simulink model "snap_adc5g_spec_rpi"  (R2019a)
settings: Solver=VariableStepDiscrete  StartTime=0.0  StopTime=10.0  RelTol=1e-3
undefined symbols (not defined in the file): pfb_coeff_gen_calc
libraries: xbsIndex_r4 x13965, casper_library_misc x80, casper_library_delays x43, xps_library x5, xbsReplacements_r4 x2, casper_library_communications x1
(part 36 of 152)

== system snap_adc5g_spec_rpi/fft_wideband_real/fft_direct/butterfly1_0/twiddle ==
  ai : Inport
  bi : Inport  Port=2
  sync_in : Inport  Port=3
  bus_convert : Subsystem  AncestorBlock=casper_library_bus/bus_convert  mask(bus_convert){n_bits_in=repmat(input_bit_width+coeff_bit_width+1, 1, n_inputs), bin_pt_in=(bin_pt_in+coeff_bit_width-1), cmplx=on, n_bits_out=input_bit_width+1, bin_pt_out=bin_pt_in, quantization=2, overflow=0, csp_latency=conv_latency, of=off, misc=on}
      mask prompts: n_bits_in "input bit widths"; bin_pt_in "input binary points"; cmplx "input complex"; n_bits_out "output bit widths"; bin_pt_out "output binary points"; quantization "quantization strategy (Truncate=0, Round  (unbiased: +/- Inf)=1, Round (unbiased: Even Values)=2)"; overflow "overflow strategy (Wrap=0, Saturate=1, Flag as error=2)"; csp_latency "latency"; of "overflow indication"; misc "misc support"
      mask help: Convert components of busses
      mask init: same as snap_adc5g_spec_rpi/fft_wideband_real/fft_direct/butterfly0_0/bus_convert
  bus_create : Subsystem  AncestorBlock=casper_library_flow_control/bus_create  mask(bus_create){inputNum=3}
      mask prompts: inputNum "Number of inputs:"
      mask init:
      | bus_create_init(gcb,...
      |     'inputNum', inputNum);
  bus_expand : Subsystem  AncestorBlock=casper_library_flow_control/bus_expand  mask(bus_expand){mode=divisions of arbitrary size, outputNum=1, outputWidth=[n_inputs*input_bit_width*2, 1+(n_inputs*input_bit_width*2)], outputBinaryPt=[0 0], outputArithmeticType=[0 0], show_format=off, outputToWorkspace=off, variablePrefix=out, outputToModelAsWell=on}
      mask prompts: outputNum "Number of outputs:"; outputWidth "Output width [msb ... lsb]:"; outputBinaryPt "Output binary point position [msb ... lsb]:"; outputArithmeticType "Output arithmetic type (ufix=0, fix=1, bool=2) [msb ... lsb]:"; show_format "Print format string?"; outputToWorkspace "Output to workspace?"; variablePrefix "Variable name prefix:"; outputToModelAsWell "Output to model as well?"
      mask help:
      | Expands a 'bus' made using a bus_create or Xilinx
      | concat block.
      | The input will be divided into the specified number
      | of outputs with the specified arithmetic types.
      | Divisions are made from most significant bit.
      mask init: same as snap_adc5g_spec_rpi/ss_adc/ctrl_split
      settings: AttributesFormatString=2 outputs
      mask TypeOptions mode: divisions of equal size | divisions of arbitrary size
      mask Callback mode: bus_expand_callback();
      mask Callback outputWidth: bus_expand_callback();
      mask Callback outputToWorkspace: bus_expand_callback();
  bus_expand1 : Subsystem  AncestorBlock=casper_library_flow_control/bus_expand  mask(bus_expand){mode=divisions of arbitrary size, outputNum=1, outputWidth=[1 72], outputBinaryPt=[0 0], outputArithmeticType=[2 0], show_format=off, outputToWorkspace=off, variablePrefix=out, outputToModelAsWell=on}
      mask prompts: outputNum "Number of outputs:"; outputWidth "Output width [msb ... lsb]:"; outputBinaryPt "Output binary point position [msb ... lsb]:"; outputArithmeticType "Output arithmetic type (ufix=0, fix=1, bool=2) [msb ... lsb]:"; show_format "Print format string?"; outputToWorkspace "Output to workspace?"; variablePrefix "Variable name prefix:"; outputToModelAsWell "Output to model as well?"
      mask help:
      | Expands a 'bus' made using a bus_create or Xilinx
      | concat block.
      | The input will be divided into the specified number
      | of outputs with the specified arithmetic types.
      | Divisions are made from most significant bit.
      mask init: same as snap_adc5g_spec_rpi/ss_adc/ctrl_split
      settings: AttributesFormatString=2 outputs
      mask TypeOptions mode: divisions of equal size | divisions of arbitrary size
      mask Callback mode: bus_expand_callback();
      mask Callback outputWidth: bus_expand_callback();
      mask Callback outputToWorkspace: bus_expand_callback();
  bus_mult : Subsystem  AncestorBlock=casper_library_bus/bus_mult  mask(bus_mult){n_bits_a=coeff_bit_width, bin_pt_a=coeff_bit_width-1, type_a=1, cmplx_a=on, n_bits_b=[18 18], bin_pt_b=bin_pt_in, type_b=1, cmplx_b=on, misc=on, floating_point=off, float_type=single, input_vec_a=1, input_vec_b=1, frac_width=24, exp_width=8, n_bits_out=input_bit_width+coeff_bit_width+1, bin_pt_out=(bin_pt_in+coeff_bit_width-1), type_out=1, quantization=0, overflow=0, mult_latency=mult_latency, add_latency=add_latency, conv_latency=0, max_fanout=max_fanout, fan_latency=2, multiplier_implementation=behavioral HDL, pipeline_cmult_en=off, pipeline_latency=0}
      mask prompts: n_bits_a "a input bit widths"; bin_pt_a "a input binary points"; type_a "a input type (Unsigned=0, Signed=1)"; cmplx_a "a input complex"; n_bits_b "b input bit widths"; bin_pt_b "b input binary points"; type_b "b input type (Unsigned=0, Signed=1)"; cmplx_b "b input complex"; misc "misc support"; floating_point "floating point"; float_type "float type"; input_vec_a "a input vector in bus"; input_vec_b "b input vector in bus"; frac_width "fraction width"; exp_width "exponent width"; n_bits_out "output bit widths"; bin_pt_out "output binary points"; type_out "output type (Unsigned=0, Signed=1)"; quantization "quantization strategy (Truncate=0, Round  (unbiased: +/- Inf)=1)"; overflow "overflow strategy (Wrap=0, Saturate=1, Flag as error=2)"; mult_latency "multiplier latency"; add_latency "adder latency"; conv_latency "convert latency"; max_fanout "limit fanout to ?"; fan_latency "fanout register latency"; multiplier_implementation "multiplier implementation"; pipeline_cmult_en "pipeline complex mult"; pipeline_latency "pipeline latency"
      mask help: Multiply components of two busses
      mask init: same as snap_adc5g_spec_rpi/fft_wideband_real/fft_direct/butterfly0_0/twiddle/bus_mult
      mask Callback floating_point:
      | onoff = get_param(gcb, 'floating_point');
      | if strcmp(onoff,'on')
      |     enable_fixpt = 'off';
      |     set_param_state(gcb, 'float_type', 'on')
      | 
      |     set_param_state(gcb, 'input_vec_a', 'on')
      |     set_param_state(gcb, 'input_vec_b', 'on')
      | 
      |     f_type = get_param(gcb, 'float_type');
      |     if strcmp(f_type,'custom')
      |         set_param_state(gcb, 'exp_width', 'on')
      |         set_param_state(gcb, 'frac_width', 'on')
      |     else
      |         set_param_state(gcb, 'exp_width', 'off')
      |         set_param_state(gcb, 'frac_width', 'off')
      |     end
      | 
      | else
      |     enable_fixpt = 'on';
      |     set_param_state(gcb, 'float_type', 'off')
      |     set_param_state(gcb, 'exp_width', 'off')
      |     set_param_state(gcb, 'frac_width', 'off')
      |     set_param_state(gcb, 'input_vec_a', 'off')
      |     set_param_state(gcb, 'input_vec_b', 'off')
      | end
      | 
      | set_param_state(gcb, 'n_bits_a', enable_fixpt)
      | set_param_state(gcb, 'bin_pt_a', enable_fixpt)
      | set_param_state(gcb, 'type_a', enable_fixpt)
      | set_param_state(gcb, 'n_bits_b', enable_fixpt)
      | set_param_state(gcb, 'bin_pt_b', enable_fixpt)
      | set_param_state(gcb, 'type_b', enable_fixpt)
      | 
      | set_param_state(gcb, 'n_bits_out', enable_fixpt)
      | set_param_state(gcb, 'bin_pt_out', enable_fixpt)
      | set_param_state(gcb, 'type_out', enable_fixpt)
      | set_param_state(gcb, 'quantization', enable_fixpt)
      | set_param_state(gcb, 'overflow', enable_fixpt)
      mask TypeOptions float_type: single | custom
      mask Callback float_type:
      | f_type = get_param(gcb, 'float_type');
      | if strcmp(f_type,'custom')
      |     set_param_state(gcb, 'exp_width', 'on')
      |     set_param_state(gcb, 'frac_width', 'on')
      | else
      |     set_param_state(gcb, 'exp_width', 'off')
      |     set_param_state(gcb, 'frac_width', 'off')
      | end
      mask TypeOptions multiplier_implementation: behavioral HDL | standard core | embedded multiplier core
      mask Callback pipeline_cmult_en:
      | pipeline_en = get_param(gcb, 'pipeline_cmult_en');
      | if strcmp(pipeline_en,'on')
      | 
      |     set_param_state(gcb, 'pipeline_latency', 'on')
      | else
      |     set_param_state(gcb, 'pipeline_latency', 'off')
      | end
  coeff_gen : Subsystem  AncestorBlock=casper_library_ffts_twiddle_coeff_gen/coeff_gen  mask(coeff_gen){FFTSize=FFTSize, Coeffs=[0 2048 1024 3072 512 2560 1536 3584 256 2304 1280 3328 768 2816 1792 3840 128 2176 1152 3200 640 2688 1664 3712 384 2432 1408 3456 896 2944 1920 3968 64 2112 1088 3136 576 2624 1600 3648 320 2368 1344 3392 832 2880 1856 3904 192 2240 1216 3264 704 2752 1728 3776 448 2496 1472 3520 960 3008 1984 4032 32 2080 1056 3104 544 2592 1568 3616 288 2336 1312 3360 800 2848 1824 3872 160 2208 1184 3232 672 2720 1696 3744 416 2464 1440 3488 928 2976 1952 4000 96 2144 1120 3168 608 2656 1632 3680 352 2400 1376 3424 864 2912 1888 3936 224 2272 1248 3296 736 2784 1760 3808 480 2528 1504 3552 992 3040 2016 4064 16 2064 1040 3088 528 2576 1552 3600 272 2320 1296 3344 784 2832 1808 3856 144 2192 1168 3216 656 2704 1680 3728 400 2448 1424 3472 912 2960 1936 3984 80 2128 1104 3152 592 2640 1616 3664 336 2384 1360 3408 848 2896 1872 3920 208 2256 1232 3280 720 2768 1744 3792 464 2512 1488 3536 976 3024 2000 4048 48 2096 1072 3120 560 2608 1584 3632 304 2352 1328 3376 816 2864 1840 3888 176 2224 1200 3248 688 2736 1712 3760 432 2480 1456 3504 944 2992 1968 4016 112 2160 1136 3184 624 2672 1648 3696 368 2416 1392 3440 880 2928 1904 3952 240 2288 1264 3312 752 2800 1776 3824 496 2544 1520 3568 1008 3056 2032 4080 8 2056 1032 3080 520 2568 1544 3592 264 2312 1288 3336 776 2824 1800 3848 136 2184 1160 3208 648 2696 1672 3720 392 2440 1416 3464 904 2952 1928 3976 72 2120 1096 3144 584 2632 1608 3656 328 2376 1352 3400 840 2888 1864 3912 200 2248 1224 3272 712 2760 1736 3784 456 2504 1480 3528 968 3016 1992 4040 40 2088 1064 3112 552 2600 1576 3624 296 2344 1320 3368 808 2856 1832 3880 168 2216 1192 3240 680 2728 1704 3752 424 2472 1448 3496 936 2984 1960 4008 104 2152 1128 3176 616 2664 1640 3688 360 2408 1384 3432 872 2920 1896 3944 232 2280 1256 3304 744 2792 1768 3816 488 2536 1512 3560 1000 3048 2024 4072 24 2072 1048 3096 536 2584 1560 3608 280 2328 1304 3352 792 2840 1816 3864 152 2200 1176 3224 664 2712 1688 3736 408 2456 1432 3480 920 2968 1944 3992 88 2136 1112 3160 600 2648 1624 3672 344 2392 1368 3416 856 2904 1880 3928 216 2264 1240 3288 728 2776 1752 3800 472 2520 1496 3544 984 3032 2008 4056 56 2104 1080 3128 568 2616 1592 3640 312 2360 1336 3384 824 2872 1848 3896 184 2232 1208 3256 696 2744 1720 3768 440 2488 1464 3512 952 3000 1976 4024 120 2168 1144 3192 632 2680 1656 3704 376 2424 1400 3448 888 2936 1912 3960 248 2296 1272 3320 760 2808 1784 3832 504 2552 1528 3576 1016 3064 2040 4088 4 2052 1028 3076 516 2564 1540 3588 260 2308 1284 3332 772 2820 1796 3844 132 2180 1156 3204 644 2692 1668 3716 388 2436 1412 3460 900 2948 1924 3972 68 2116 1092 3140 580 2628 1604 3652 324 2372 1348 3396 836 2884 1860 3908 196 2244 1220 3268 708 2756 1732 3780 452 2500 1476 3524 964 3012 1988 4036 36 2084 1060 3108 548 2596 1572 3620 292 2340 1316 3364 804 2852 1828 3876 164 2212 1188 3236 676 2724 1700 3748 420 2468 1444 3492 932 2980 1956 4004 100 2148 1124 3172 612 2660 1636 3684 356 2404 1380 3428 868 2916 1892 3940 228 2276 1252 3300 740 2788 1764 3812 484 2532 1508 3556 996 3044 2020 4068 20 2068 1044 3092 532 2580 1556 3604 276 2324 1300 3348 788 2836 1812 3860 148 2196 1172 3220 660 2708 1684 3732 404 2452 1428 3476 916 2964 1940 3988 84 2132 1108 3156 596 2644 1620 3668 340 2388 1364 3412 852 2900 1876 3924 212 2260 1236 3284 724 2772 1748 3796 468 2516 1492 3540 980 3028 2004 4052 52 2100 1076 3124 564 2612 1588 3636 308 2356 1332 3380 820 2868 1844 3892 180 2228 1204 3252 692 2740 1716 3764 436 2484 1460 3508 948 2996 1972 4020 116 2164 1140 3188 628 2676 1652 3700 372 2420 1396 3444 884 2932 1908 3956 244 2292 1268 3316 756 2804 1780 3828 500 2548 1524 3572 1012 3060 2036 4084 12 2060 1036 3084 524 2572 1548 3596 268 2316 1292 3340 780 2828 1804 3852 140 2188 1164 3212 652 2700 1676 3724 396 2444 1420 3468 908 2956 1932 3980 76 2124 1100 3148 588 2636 1612 3660 332 2380 1356 3404 844 2892 1868 3916 204 2252 1228 3276 716 2764 1740 3788 460 2508 1484 3532 972 3020 1996 4044 44 2092 1068 3116 556 2604 1580 3628 300 2348 1324 3372 812 2860 ...(+5688 chars)], coeff_bit_width=coeff_bit_width, StepPeriod=StepPeriod, async=off, misc=on, floating_point=off, float_type=single, exp_width=8, frac_width=24, bram_latency=bram_latency, mult_latency=mult_latency, add_latency=add_latency, conv_latency=conv_latency, coeffs_bit_limit=coeffs_bit_limit, coeff_sharing=on, coeff_decimation=on, coeff_generation=off, cal_bits=cal_bits, n_bits_rotation=n_bits_rotation, quantization=Round  (unbiased: Even Values)}
      mask prompts: FFTSize "fft size (2^?)"; Coeffs "Coefficients"; coeff_bit_width "Coefficient Bit Width:"; StepPeriod "Step Period: (2^?)"; async "asynchronous operation"; misc "misc port"; floating_point "floating point"; exp_width "exponential width"; frac_width "fractional width"; bram_latency "BRAM latency"; mult_latency "Multiplier latency"; add_latency "Adder latency"; conv_latency "Convert latency"; coeffs_bit_limit "Number bits above which to store stage's coefficients in BRAM (2^? bits)"; coeff_sharing "BRAM sharing in coeff storage"; coeff_decimation "Store a fraction of coeff factors where useful"; coeff_generation "Generate coeffs with multipliers where useful"; cal_bits "Number calibration locations when generating coeffs (2^?)"; n_bits_rotation "Rotation vector resolution"; quantization "Quantization strategy"
      mask help:
      | Generates a sequence of complex coefficients for use in generating twiddle
      | factors for FFTs.
      mask init: same as snap_adc5g_spec_rpi/fft_wideband_real/fft_direct/butterfly0_0/twiddle/coeff_gen
      settings: AttributesFormatString=2048 @ (18,17)
      mask Callback floating_point:
      | onoff = get_param(gcb, 'floating_point');
      | if strcmp(onoff,'on')
      |     enable_fixpt = 'off'
      |     set_param_state(gcb, 'float_type', 'on')
      | 
      |     f_type = get_param(gcb, 'float_type')
      |     if strcmp(f_type,'custom')
      |         set_param_state(gcb, 'exp_width', 'on')
      |         set_param_state(gcb, 'frac_width', 'on')
      |     else
      |         set_param_state(gcb, 'exp_width', 'off')
      |         set_param_state(gcb, 'frac_width', 'off')
      |     end
      | 
      | 
      | else
      |     enable_fixpt = 'on'
      |     set_param_state(gcb, 'float_type', 'off')
      |     set_param_state(gcb, 'exp_width', 'off')
      |     set_param_state(gcb, 'frac_width', 'off')
      | end
      mask TypeOptions float_type: single | custom
      mask Callback float_type:
      | f_type = get_param(gcb, 'float_type')
      | if strcmp(f_type,'custom')
      |     set_param_state(gcb, 'exp_width', 'on')
      |     set_param_state(gcb, 'frac_width', 'on')
      | else
      |     set_param_state(gcb, 'exp_width', 'off')
      |     set_param_state(gcb, 'frac_width', 'off')
      | end
      mask TypeOptions quantization: Truncate | Round  (unbiased: +/- Inf) | Round  (unbiased: Even Values)
      mask DialogControl ParameterTabVar0 Prompt: basic
      mask DialogControl ParameterTabVar01 Prompt: latency
      mask DialogControl ParameterTabVar012 Prompt: implementation
  ao : Outport
  bwo : Outport  Port=2
  sync_out : Outport  Port=3
  wires:
  bi/1 -> bus_create/1(in1)
  sync_in/1 -> bus_create/2(in2), coeff_gen/1(rst)
  ai/1 -> bus_create/3(in3)
  bus_create/1(bus_out) -> coeff_gen/2(misci)
  coeff_gen/2(misco) -> bus_expand/1(bus_in)
  coeff_gen/1(w) -> bus_mult/1(a)
  bus_expand/2(lsb_out1) -> bus_mult/3(misci)
  bus_expand/1(msb_out2) -> bus_mult/2(b)
  bus_mult/1(a*b) -> bus_convert/1(din)
  bus_mult/2(misco) -> bus_convert/2(misci)
  bus_convert/1(dout) -> bwo/1
  bus_convert/2(misco) -> bus_expand1/1(bus_in)
  bus_expand1/1(msb_out2) -> sync_out/1
  bus_expand1/2(lsb_out1) -> ao/1

== system snap_adc5g_spec_rpi/fft_wideband_real/fft_direct/butterfly1_1/bus_add ==
  a : Inport
  b : Inport  Port=2
  a_debus : Subsystem  AncestorBlock=casper_library_flow_control/bus_expand  mask(bus_expand){mode=divisions of arbitrary size, outputNum=1, outputWidth=[18  18  18  18], outputBinaryPt=[17  17  17  17], outputArithmeticType=[1  1  1  1], show_format=on, outputToWorkspace=off, variablePrefix=, outputToModelAsWell=on}
      mask prompts: outputNum "Number of outputs:"; outputWidth "Output width [msb ... lsb]:"; outputBinaryPt "Output binary point position [msb ... lsb]:"; outputArithmeticType "Output arithmetic type (ufix=0, fix=1, bool=2) [msb ... lsb]:"; show_format "Print format string?"; outputToWorkspace "Output to workspace?"; variablePrefix "Variable name prefix:"; outputToModelAsWell "Output to model as well?"
      mask help:
      | Expands a 'bus' made using a bus_create or Xilinx
      | concat block.
      | The input will be divided into the specified number
      | of outputs with the specified arithmetic types.
      | Divisions are made from most significant bit.
      mask init: same as snap_adc5g_spec_rpi/ss_adc/ctrl_split
      settings: AttributesFormatString=4 outputs: f18.17,f18.17,f18.17,f18.17,
      mask TypeOptions mode: divisions of equal size | divisions of arbitrary size
      mask Callback mode: bus_expand_callback();
      mask Callback outputWidth: bus_expand_callback();
      mask Callback outputToWorkspace: bus_expand_callback();
  addsub{1..4} (4 alike) : xbsIndex_r4/AddSub  mode=Addition  use_carryin=off  use_carryout=off  en=off  latency=1  precision=User Defined  arith_type="Signed  (2's comp)"  n_bits=20  bin_pt=17  quantization=Truncate  overflow=Wrap  use_behavioral_HDL=on  hw_selection=Fabric  pipelined=on  dbl_ovrd=off  block_type=addsub
  b_debus : Subsystem  AncestorBlock=casper_library_flow_control/bus_expand  mask(bus_expand){mode=divisions of arbitrary size, outputNum=1, outputWidth=[19  19  19  19], outputBinaryPt=[17  17  17  17], outputArithmeticType=[1  1  1  1], show_format=on, outputToWorkspace=off, variablePrefix=, outputToModelAsWell=on}
      mask prompts: outputNum "Number of outputs:"; outputWidth "Output width [msb ... lsb]:"; outputBinaryPt "Output binary point position [msb ... lsb]:"; outputArithmeticType "Output arithmetic type (ufix=0, fix=1, bool=2) [msb ... lsb]:"; show_format "Print format string?"; outputToWorkspace "Output to workspace?"; variablePrefix "Variable name prefix:"; outputToModelAsWell "Output to model as well?"
      mask help:
      | Expands a 'bus' made using a bus_create or Xilinx
      | concat block.
      | The input will be divided into the specified number
      | of outputs with the specified arithmetic types.
      | Divisions are made from most significant bit.
      mask init: same as snap_adc5g_spec_rpi/ss_adc/ctrl_split
      settings: AttributesFormatString=4 outputs: f19.17,f19.17,f19.17,f19.17,
      mask TypeOptions mode: divisions of equal size | divisions of arbitrary size
      mask Callback mode: bus_expand_callback();
      mask Callback outputWidth: bus_expand_callback();
      mask Callback outputToWorkspace: bus_expand_callback();
  op_bussify : Subsystem  AncestorBlock=casper_library_flow_control/bus_create  mask(bus_create){inputNum=4}
      mask prompts: inputNum "Number of inputs:"
      mask init:
      | bus_create_init(gcb,...
      |     'inputNum', inputNum);
  dout : Outport
  wires:
  a/1 -> a_debus/1(bus_in)
  b/1 -> b_debus/1(bus_in)
  a_debus/1(msb_out4) -> addsub1/1
  b_debus/1(msb_out4) -> addsub1/2
  a_debus/2(out3) -> addsub2/1
  b_debus/2(out3) -> addsub2/2
  a_debus/3(out2) -> addsub3/1
  b_debus/3(out2) -> addsub3/2
  a_debus/4(lsb_out1) -> addsub4/1
  b_debus/4(lsb_out1) -> addsub4/2
  addsub1/1 -> op_bussify/1(in1)
  addsub2/1 -> op_bussify/2(in2)
  addsub3/1 -> op_bussify/3(in3)
  addsub4/1 -> op_bussify/4(in4)
  op_bussify/1(bus_out) -> dout/1

== system snap_adc5g_spec_rpi/fft_wideband_real/fft_direct/butterfly1_1/bus_convert ==
  din : Inport
  bussify : Subsystem  AncestorBlock=casper_library_flow_control/bus_create  mask(bus_create){inputNum=8}
      mask prompts: inputNum "Number of inputs:"
      mask init:
      | bus_create_init(gcb,...
      |     'inputNum', inputNum);
  conv1 : Subsystem  AncestorBlock=casper_library_misc/convert_of  mask(convert_of){bit_width_i=21, binary_point_i=18, bit_width_o=18, binary_point_o=17, csp_latency=1, overflow=Wrap, quantization=Round  (unbiased: even values)}
      mask prompts: bit_width_i "Bit Width In"; binary_point_i "Binary Point In"; bit_width_o "Bit Width Out"; binary_point_o "Binary Point Out"; csp_latency "Latency"; overflow "Overflow Behaviour"; quantization "Quantization Behaviour"
      mask help:
      | Converts from one 2's complement bit-width
      | and/or binary point position to another.
      | Includes underflow/overflow indicator.
      mask init: same as snap_adc5g_spec_rpi/fft_wideband_real/fft_direct/butterfly0_0/bus_convert/conv1
      settings: AttributesFormatString=[21,18]->[18,17]
      mask TypeOptions overflow: Wrap | Saturate | Error
      mask TypeOptions quantization: Truncate | Round  (unbiased: +/- Inf) | Round  (unbiased: even values)
  conv2 : Subsystem  AncestorBlock=casper_library_misc/convert_of  mask(convert_of){bit_width_i=21, binary_point_i=18, bit_width_o=18, binary_point_o=17, csp_latency=1, overflow=Wrap, quantization=Round  (unbiased: even values)}
      mask prompts: bit_width_i "Bit Width In"; binary_point_i "Binary Point In"; bit_width_o "Bit Width Out"; binary_point_o "Binary Point Out"; csp_latency "Latency"; overflow "Overflow Behaviour"; quantization "Quantization Behaviour"
      mask help:
      | Converts from one 2's complement bit-width
      | and/or binary point position to another.
      | Includes underflow/overflow indicator.
      mask init: same as snap_adc5g_spec_rpi/fft_wideband_real/fft_direct/butterfly0_0/bus_convert/conv1
      settings: AttributesFormatString=[21,18]->[18,17]
      mask TypeOptions overflow: Wrap | Saturate | Error
      mask TypeOptions quantization: Truncate | Round  (unbiased: +/- Inf) | Round  (unbiased: even values)
  conv3 : Subsystem  AncestorBlock=casper_library_misc/convert_of  mask(convert_of){bit_width_i=21, binary_point_i=18, bit_width_o=18, binary_point_o=17, csp_latency=1, overflow=Wrap, quantization=Round  (unbiased: even values)}
      mask prompts: bit_width_i "Bit Width In"; binary_point_i "Binary Point In"; bit_width_o "Bit Width Out"; binary_point_o "Binary Point Out"; csp_latency "Latency"; overflow "Overflow Behaviour"; quantization "Quantization Behaviour"
      mask help:
      | Converts from one 2's complement bit-width
      | and/or binary point position to another.
      | Includes underflow/overflow indicator.
      mask init: same as snap_adc5g_spec_rpi/fft_wideband_real/fft_direct/butterfly0_0/bus_convert/conv1
      settings: AttributesFormatString=[21,18]->[18,17]
      mask TypeOptions overflow: Wrap | Saturate | Error
      mask TypeOptions quantization: Truncate | Round  (unbiased: +/- Inf) | Round  (unbiased: even values)
  conv4 : Subsystem  AncestorBlock=casper_library_misc/convert_of  mask(convert_of){bit_width_i=21, binary_point_i=18, bit_width_o=18, binary_point_o=17, csp_latency=1, overflow=Wrap, quantization=Round  (unbiased: even values)}
      mask prompts: bit_width_i "Bit Width In"; binary_point_i "Binary Point In"; bit_width_o "Bit Width Out"; binary_point_o "Binary Point Out"; csp_latency "Latency"; overflow "Overflow Behaviour"; quantization "Quantization Behaviour"
      mask help:
      | Converts from one 2's complement bit-width
      | and/or binary point position to another.
      | Includes underflow/overflow indicator.
      mask init: same as snap_adc5g_spec_rpi/fft_wideband_real/fft_direct/butterfly0_0/bus_convert/conv1
      settings: AttributesFormatString=[21,18]->[18,17]
      mask TypeOptions overflow: Wrap | Saturate | Error
      mask TypeOptions quantization: Truncate | Round  (unbiased: +/- Inf) | Round  (unbiased: even values)
  conv5 : Subsystem  AncestorBlock=casper_library_misc/convert_of  mask(convert_of){bit_width_i=21, binary_point_i=18, bit_width_o=18, binary_point_o=17, csp_latency=1, overflow=Wrap, quantization=Round  (unbiased: even values)}
      mask prompts: bit_width_i "Bit Width In"; binary_point_i "Binary Point In"; bit_width_o "Bit Width Out"; binary_point_o "Binary Point Out"; csp_latency "Latency"; overflow "Overflow Behaviour"; quantization "Quantization Behaviour"
      mask help:
      | Converts from one 2's complement bit-width
      | and/or binary point position to another.
      | Includes underflow/overflow indicator.
      mask init: same as snap_adc5g_spec_rpi/fft_wideband_real/fft_direct/butterfly0_0/bus_convert/conv1
      settings: AttributesFormatString=[21,18]->[18,17]
      mask TypeOptions overflow: Wrap | Saturate | Error
      mask TypeOptions quantization: Truncate | Round  (unbiased: +/- Inf) | Round  (unbiased: even values)
  conv6 : Subsystem  AncestorBlock=casper_library_misc/convert_of  mask(convert_of){bit_width_i=21, binary_point_i=18, bit_width_o=18, binary_point_o=17, csp_latency=1, overflow=Wrap, quantization=Round  (unbiased: even values)}
      mask prompts: bit_width_i "Bit Width In"; binary_point_i "Binary Point In"; bit_width_o "Bit Width Out"; binary_point_o "Binary Point Out"; csp_latency "Latency"; overflow "Overflow Behaviour"; quantization "Quantization Behaviour"
      mask help:
      | Converts from one 2's complement bit-width
      | and/or binary point position to another.
      | Includes underflow/overflow indicator.
      mask init: same as snap_adc5g_spec_rpi/fft_wideband_real/fft_direct/butterfly0_0/bus_convert/conv1
      settings: AttributesFormatString=[21,18]->[18,17]
      mask TypeOptions overflow: Wrap | Saturate | Error
      mask TypeOptions quantization: Truncate | Round  (unbiased: +/- Inf) | Round  (unbiased: even values)
  conv7 : Subsystem  AncestorBlock=casper_library_misc/convert_of  mask(convert_of){bit_width_i=21, binary_point_i=18, bit_width_o=18, binary_point_o=17, csp_latency=1, overflow=Wrap, quantization=Round  (unbiased: even values)}
      mask prompts: bit_width_i "Bit Width In"; binary_point_i "Binary Point In"; bit_width_o "Bit Width Out"; binary_point_o "Binary Point Out"; csp_latency "Latency"; overflow "Overflow Behaviour"; quantization "Quantization Behaviour"
      mask help:
      | Converts from one 2's complement bit-width
      | and/or binary point position to another.
      | Includes underflow/overflow indicator.
      mask init: same as snap_adc5g_spec_rpi/fft_wideband_real/fft_direct/butterfly0_0/bus_convert/conv1
      settings: AttributesFormatString=[21,18]->[18,17]
      mask TypeOptions overflow: Wrap | Saturate | Error
      mask TypeOptions quantization: Truncate | Round  (unbiased: +/- Inf) | Round  (unbiased: even values)
  conv8 : Subsystem  AncestorBlock=casper_library_misc/convert_of  mask(convert_of){bit_width_i=21, binary_point_i=18, bit_width_o=18, binary_point_o=17, csp_latency=1, overflow=Wrap, quantization=Round  (unbiased: even values)}
      mask prompts: bit_width_i "Bit Width In"; binary_point_i "Binary Point In"; bit_width_o "Bit Width Out"; binary_point_o "Binary Point Out"; csp_latency "Latency"; overflow "Overflow Behaviour"; quantization "Quantization Behaviour"
      mask help:
      | Converts from one 2's complement bit-width
      | and/or binary point position to another.
      | Includes underflow/overflow indicator.
      mask init: same as snap_adc5g_spec_rpi/fft_wideband_real/fft_direct/butterfly0_0/bus_convert/conv1
      settings: AttributesFormatString=[21,18]->[18,17]
      mask TypeOptions overflow: Wrap | Saturate | Error
      mask TypeOptions quantization: Truncate | Round  (unbiased: +/- Inf) | Round  (unbiased: even values)
  debus : Subsystem  AncestorBlock=casper_library_flow_control/bus_expand  mask(bus_expand){mode=divisions of arbitrary size, outputNum=1, outputWidth=[21 21 21 21 21 21 21 21], outputBinaryPt=[18 18 18 18 18 18 18 18], outputArithmeticType=[1 1 1 1 1 1 1 1], show_format=on, outputToWorkspace=off, variablePrefix=, outputToModelAsWell=on}
      mask prompts: outputNum "Number of outputs:"; outputWidth "Output width [msb ... lsb]:"; outputBinaryPt "Output binary point position [msb ... lsb]:"; outputArithmeticType "Output arithmetic type (ufix=0, fix=1, bool=2) [msb ... lsb]:"; show_format "Print format string?"; outputToWorkspace "Output to workspace?"; variablePrefix "Variable name prefix:"; outputToModelAsWell "Output to model as well?"
      mask help:
      | Expands a 'bus' made using a bus_create or Xilinx
      | concat block.
      | The input will be divided into the specified number
      | of outputs with the specified arithmetic types.
      | Divisions are made from most significant bit.
      mask init: same as snap_adc5g_spec_rpi/ss_adc/ctrl_split
      settings: AttributesFormatString=8 outputs: f21.18,f21.18,f21.18,f21.18,f21.18,f21.18,f21.18,f21.18,
      mask TypeOptions mode: divisions of equal size | divisions of arbitrary size
      mask Callback mode: bus_expand_callback();
      mask Callback outputWidth: bus_expand_callback();
      mask Callback outputToWorkspace: bus_expand_callback();
  of_bussify : Subsystem  AncestorBlock=casper_library_flow_control/bus_create  mask(bus_create){inputNum=8}
      mask prompts: inputNum "Number of inputs:"
      mask init:
      | bus_create_init(gcb,...
      |     'inputNum', inputNum);
  dout : Outport
  overflow : Outport  Port=2
  wires:
  din/1 -> debus/1(bus_in)
  debus/1(msb_out8) -> conv1/1(din)
  debus/2(out7) -> conv2/1(din)
  debus/3(out6) -> conv3/1(din)
  debus/4(out5) -> conv4/1(din)
  debus/5(out4) -> conv5/1(din)
  debus/6(out3) -> conv6/1(din)
  debus/7(out2) -> conv7/1(din)
  debus/8(lsb_out1) -> conv8/1(din)
  conv1/1(dout) -> bussify/1(in1)
  conv2/1(dout) -> bussify/2(in2)
  conv3/1(dout) -> bussify/3(in3)
  conv4/1(dout) -> bussify/4(in4)
  conv5/1(dout) -> bussify/5(in5)
  conv6/1(dout) -> bussify/6(in6)
  conv7/1(dout) -> bussify/7(in7)
  conv8/1(dout) -> bussify/8(in8)
  conv1/2(of) -> of_bussify/1(in1)
  conv2/2(of) -> of_bussify/2(in2)
  conv3/2(of) -> of_bussify/3(in3)
  conv4/2(of) -> of_bussify/4(in4)
  conv5/2(of) -> of_bussify/5(in5)
  conv6/2(of) -> of_bussify/6(in6)
  conv7/2(of) -> of_bussify/7(in7)
  conv8/2(of) -> of_bussify/8(in8)
  bussify/1(bus_out) -> dout/1
  of_bussify/1(bus_out) -> overflow/1

== system snap_adc5g_spec_rpi/fft_wideband_real/fft_direct/butterfly1_1/bus_expand ==
  bus_in : Inport
  reinterpret1 : xbsIndex_r4/Reinterpret  force_arith_type=on  arith_type=Unsigned  force_bin_pt=on  bin_pt=0  block_type=reinterpret
  reinterpret2 : xbsIndex_r4/Reinterpret  force_arith_type=on  arith_type=Unsigned  force_bin_pt=on  bin_pt=0  block_type=reinterpret
  slice1 : xbsIndex_r4/Slice  nbits=72  boolean_output=off  mode=Upper Bit Location + Width  bit1=-72  base1=MSB of Input  bit0=0  base0=LSB of Input  dbl_ovrd=off  block_type=slice
  slice2 : xbsIndex_r4/Slice  nbits=72  boolean_output=off  mode=Upper Bit Location + Width  bit1=0  base1=MSB of Input  bit0=0  base0=LSB of Input  dbl_ovrd=off  block_type=slice
  msb_out2 : Outport
  lsb_out1 : Outport  Port=2
  wires:
  bus_in/1 -> slice2/1, slice1/1
  slice2/1 -> reinterpret2/1
  reinterpret2/1 -> msb_out2/1
  slice1/1 -> reinterpret1/1
  reinterpret1/1 -> lsb_out1/1

== system snap_adc5g_spec_rpi/fft_wideband_real/fft_direct/butterfly1_1/bus_norm0 ==
  din : Inport
  bussify : Subsystem  AncestorBlock=casper_library_flow_control/bus_create  mask(bus_create){inputNum=8}
      mask prompts: inputNum "Number of inputs:"
      mask init:
      | bus_create_init(gcb,...
      |     'inputNum', inputNum);
  conv{1..8} (8 alike) : xbsIndex_r4/Convert  gui_display_data_type=Fixed-point  arith_type="Signed  (2's comp)"  n_bits=21  bin_pt=18  float_type=Single  exp_bits=8  fraction_bits=24  quantization=Truncate  overflow=Wrap  en=off  latency=0  pipeline=on  dbl_ovrd=off  block_type=convert
  debus : Subsystem  AncestorBlock=casper_library_flow_control/bus_expand  mask(bus_expand){mode=divisions of arbitrary size, outputNum=1, outputWidth=[20 20 20 20 20 20 20 20], outputBinaryPt=[17 17 17 17 17 17 17 17], outputArithmeticType=[1 1 1 1 1 1 1 1], show_format=on, outputToWorkspace=off, variablePrefix=, outputToModelAsWell=on}
      mask prompts: outputNum "Number of outputs:"; outputWidth "Output width [msb ... lsb]:"; outputBinaryPt "Output binary point position [msb ... lsb]:"; outputArithmeticType "Output arithmetic type (ufix=0, fix=1, bool=2) [msb ... lsb]:"; show_format "Print format string?"; outputToWorkspace "Output to workspace?"; variablePrefix "Variable name prefix:"; outputToModelAsWell "Output to model as well?"
      mask help:
      | Expands a 'bus' made using a bus_create or Xilinx
      | concat block.
      | The input will be divided into the specified number
      | of outputs with the specified arithmetic types.
      | Divisions are made from most significant bit.
      mask init: same as snap_adc5g_spec_rpi/ss_adc/ctrl_split
      settings: AttributesFormatString=8 outputs: f20.17,f20.17,f20.17,f20.17,f20.17,f20.17,f20.17,f20.17,
      mask TypeOptions mode: divisions of equal size | divisions of arbitrary size
      mask Callback mode: bus_expand_callback();
      mask Callback outputWidth: bus_expand_callback();
      mask Callback outputToWorkspace: bus_expand_callback();
  dout : Outport
  wires:
  din/1 -> debus/1(bus_in)
  debus/1(msb_out8) -> conv1/1
  debus/2(out7) -> conv2/1
  debus/3(out6) -> conv3/1
  debus/4(out5) -> conv4/1
  debus/5(out4) -> conv5/1
  debus/6(out3) -> conv6/1
  debus/7(out2) -> conv7/1
  debus/8(lsb_out1) -> conv8/1
  conv1/1 -> bussify/1(in1)
  conv2/1 -> bussify/2(in2)
  conv3/1 -> bussify/3(in3)
  conv4/1 -> bussify/4(in4)
  conv5/1 -> bussify/5(in5)
  conv6/1 -> bussify/6(in6)
  conv7/1 -> bussify/7(in7)
  conv8/1 -> bussify/8(in8)
  bussify/1(bus_out) -> dout/1
